simulink model "tb_lv_rails"  (R2026b)
model workspace (MAT data in the model file):
  TB.vaux_t = [0 10000000]
  TB.vaux_v = [52 52]
  TB.P24_t = [0 10000000]
  TB.P24_v = [53 53]
  TB.P12_t = [0 10000000]
  TB.P12_v = [99 99]
  TB.P5_t = [0 10000000]
  TB.P5_v = [2.5 2.5]
  TB.P3_t = [0 10000000]
  TB.P3_v = [0.6 0.6]
  TB.fan_t = [0 10000000]
  TB.fan_v = [0 0]
  TB.k3_t = [0 10000000]
  TB.k3_v = [0 0]
  TB.imp_R = 1000
  TB.MaxNonlinIter = 3
  TB.MaxModeIter = 2
undefined symbols (not defined in the file or in its folder): Ts
libraries: fl_lib x4, nesl_utility x4, simulink x1, ee_lib x1
settings Model: Creator=aomar  LastModifiedBy=aomar

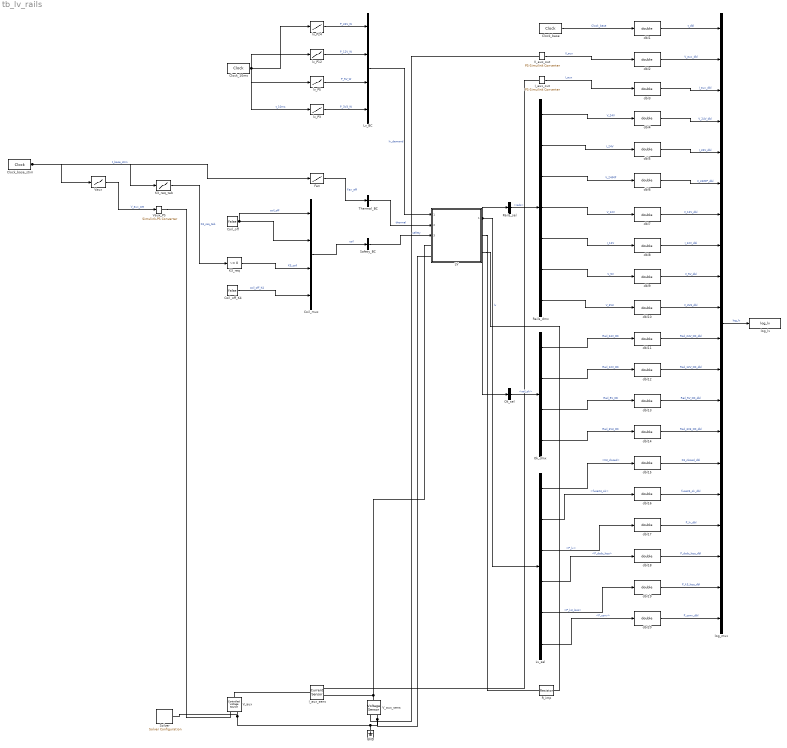
== system tb_lv_rails ==
  Clock_10ms : DigitalClock  SampleTime=Ts.ctrl
  Clock_base : DigitalClock  SampleTime=Ts.base
  Clock_base_stim : DigitalClock  SampleTime=Ts.base
  Coil_mux : Mux
  Coil_off : Constant  Value=false  OutDataTypeStr=boolean  SampleTime=Ts.base
  Coil_off_K4 : Constant  Value=false  OutDataTypeStr=boolean  SampleTime=Ts.base
  Fan : Lookup_n-D  NumberOfTableDimensions=1  BreakpointsForDimension1=TB.fan_t  Table=TB.fan_v  InterpMethod=Flat  ExtrapMethod=Clip  InternalRulePriority=Speed  RndMeth=Simplest
  GND : fl_lib/Electrical/Electrical Elements/Electrical Reference
  I_aux_out : nesl_utility/PS-Simulink Converter  PhysicalDomain=network_engine_domain  SubClassName=ps_output  LeftPortType=input  RightPortType=output  PseudoPeriodic=off  Frequencies=[]  VectorFormat=inherit  Unit=A  AffineConversion=off
  I_aux_sens : fl_lib/Electrical/Electrical Sensors/Current Sensor
  K3_req : simulink/Logic and Bit Operations/Compare To Zero  relop=~=  OutDataTypeStr=boolean
  K3_req_tab : Lookup_n-D  NumberOfTableDimensions=1  BreakpointsForDimension1=TB.k3_t  Table=TB.k3_v  InterpMethod=Flat  ExtrapMethod=Clip  InternalRulePriority=Speed  RndMeth=Simplest
  LV : Subsystem  ReferencedSubsystem=LV_Distribution
  Lv_BC : BusCreator  Inputs=4  OutDataTypeStr=Bus: Bus_LV_LoadDemand  NonVirtualBus=on
      settings: InheritFromInputs=off
  Lv_sel : BusSelector  OutputSignals=K3_closed,fuse24_ok,P_lv,P_dcdc_loss,P_k3_loss,P_conv
  Ok_dmx : Demux
  Ok_sel : BusSelector  OutputSignals=rail_ok
  R_imp : ee_lib/Passive/Resistor  R=TB.imp_R Ohm  enable_R_tol=ee.enum.toleranceApplication.none  R_tol=5  tol_distribution=ee.enum.toleranceDistribution.uniform  nSigma=4  enable_operating_limits=ee.enum.enable.no  operating_limit_action=ee.enum.passive.reportOpLim.warn  power_rating=1 W  max_working_voltage=100 V  noise_mode=ee.enum.sources.noise.Disabled  Tdevice=25 degC  sample_time=1e-3 s  repeatability=ee.enum.ic.repeatability.notRepeatable  user_seed=0  auto_seed=1503454846  power_derating_T1=70 degC  power_derating_T2=155 degC  operating_temperature_range_vec=[-50, 150] degC  alpha=3.93e-3 1/K  Tmeas=25 degC  thermal_mass=100 J/K  temperature_specify=off  temperature_priority=High  temperature=298.15 K  temperature_nominal_specify=off  temperature_nominal_value=1  temperature_nominal_unit=K
  Rails_dmx : Demux  Outputs=7
  Rails_sel : BusSelector  OutputSignals=rails
  Safety_BC : BusCreator  Inputs=1
  Solver : nesl_utility/Solver Configuration  PhysicalDomain=network_engine_domain  SubClassName=solver  LeftPortType=input  RightPortType=generic  Tones=[]  Harmonics=[]  SimulateNoise=off  Profile=off  UseLocalSampling=off  EnableSwitchedLinearOptims=on  FrequencyDomain=off  UseCCode=off  RelTol=0.001  AbsTol=0.001  MinStep=1e-09  ToWorkspace=off  RevertToSquareIcSolve=off  NumHomotopyIterations=100  PhasorMode=off  PhasorModeNumHarmonics=1  ConsistencySolver=NEWTON_XTOL_AFTER_FTOL  CanonicalOrdering=CANONICAL  OptimizeIntermediates=OPTIMIZED  MulticoreSolverChoice=BACKWARD_EULER  IndexReductionMethod=DerivativeReplacement  DoDC=off  ResidualTolerance=1e-09  ConsistencyTolSource=GLOBAL  ConsistencyAbsTol=0.001  ConsistencyRelTol=0.001  ConsistencyTolFactor=0.001  UseLocalSolver=on  LocalSolverChoice=NE_BACKWARD_EULER_ADVANCER  ResolveIndetEquations=on  FunctionEvalNumThread=1  LocalSolverSampleTime=P.sim.ssc.Ts  DoFixedCost=on  MaxNonlinIter=TB.MaxNonlinIter  MaxModeIter=TB.MaxModeIter  ComputeImpulses=off  ImpulseIterations=2  LinearAlgebra=auto  LinearAlgebraNumThread=0  EquationFormulation=NE_TIME_EF  DelaysMemoryBudget=1024  AutomaticFiltering=on  FilteringTimeConstant=0.001  PartitionStorageMethod=AS_NEEDED  PartitionMemoryBudget=1024  PartitionMethod=BALANCED  MultibodyUseLocalSolver=off  MultibodyLocalSolverChoice=ODE1  MultibodyLocalSolverSampleTime=0.001
  Thermal_BC : BusCreator  Inputs=1
  V_aux : fl_lib/Electrical/Electrical Sources/Controlled Voltage Source
  V_aux_out : nesl_utility/PS-Simulink Converter  PhysicalDomain=network_engine_domain  SubClassName=ps_output  LeftPortType=input  RightPortType=output  PseudoPeriodic=off  Frequencies=[]  VectorFormat=inherit  Unit=V  AffineConversion=off
  V_aux_sens : fl_lib/Electrical/Electrical Sensors/Voltage Sensor
  Vaux : Lookup_n-D  NumberOfTableDimensions=1  BreakpointsForDimension1=TB.vaux_t  Table=TB.vaux_v  ExtrapMethod=Clip  InternalRulePriority=Speed  RndMeth=Simplest
  Vaux_PS : nesl_utility/Simulink-PS Converter  PhysicalDomain=network_engine_domain  SubClassName=ps_input  LeftPortType=input  RightPortType=output  PseudoPeriodic=off  Frequencies=[]  NoiseDistribution=none  NoiseParameters=[]  Unit=V  AffineConversion=off  FilteringAndDerivatives=zero  SimscapeFilterOrder=1  InputFilterTimeConstant=0.001  UdotUserProvided=0
  dbl{1..20} (20 alike) : DataTypeConversion  OutDataTypeStr=double  SaturateOnIntegerOverflow=off  RndMeth=Floor
  log_lv : ToWorkspace  VariableName=log_lv  SampleTime=-1
  log_mux : Mux  Inputs=20
  lv_P12 : Lookup_n-D  NumberOfTableDimensions=1  BreakpointsForDimension1=TB.P12_t  Table=TB.P12_v  InterpMethod=Flat  ExtrapMethod=Clip  InternalRulePriority=Speed  RndMeth=Simplest
  lv_P24 : Lookup_n-D  NumberOfTableDimensions=1  BreakpointsForDimension1=TB.P24_t  Table=TB.P24_v  InterpMethod=Flat  ExtrapMethod=Clip  InternalRulePriority=Speed  RndMeth=Simplest
  lv_P3 : Lookup_n-D  NumberOfTableDimensions=1  BreakpointsForDimension1=TB.P3_t  Table=TB.P3_v  InterpMethod=Flat  ExtrapMethod=Clip  InternalRulePriority=Speed  RndMeth=Simplest
  lv_P5 : Lookup_n-D  NumberOfTableDimensions=1  BreakpointsForDimension1=TB.P5_t  Table=TB.P5_v  InterpMethod=Flat  ExtrapMethod=Clip  InternalRulePriority=Speed  RndMeth=Simplest
  wires:
  Clock_base_stim/1 -> K3_req_tab/1, Vaux/1, Fan/1  "t_base_stim"
  Vaux/1 -> Vaux_PS/1  "V_aux_set"
  K3_req_tab/1 -> K3_req/1  "K3_req_tab"
  Coil_off/1 -> Coil_mux/2, Coil_mux/1  "coil_off"
  Coil_off_K4/1 -> Coil_mux/4  "coil_off_K4"
  K3_req/1 -> Coil_mux/3  "K3_coil"
  Clock_10ms/1 -> lv_P24/1, lv_P3/1, lv_P12/1, lv_P5/1  "t_10ms"
  Coil_mux/1 -> Safety_BC/1  "coil"
  lv_P24/1 -> Lv_BC/1  "P_24V_W"
  lv_P12/1 -> Lv_BC/2  "P_12V_W"
  lv_P5/1 -> Lv_BC/3  "P_5V_W"
  lv_P3/1 -> Lv_BC/4  "P_3V3_W"
  Fan/1 -> Thermal_BC/1  "Fan_eff"
  Lv_BC/1 -> LV/1  "lv_demand"
  Thermal_BC/1 -> LV/2  "thermal"
  Safety_BC/1 -> LV/3  "safety"
  LV/1 -> Lv_sel/1, Ok_sel/1, Rails_sel/1  "lv"
  Rails_sel/1 -> Rails_dmx/1  "<rails>"
  Ok_sel/1 -> Ok_dmx/1  "<rail_ok>"
  Rails_dmx/1 -> dbl4/1  "V_24V"
  Rails_dmx/2 -> dbl5/1  "I_24V"
  Rails_dmx/3 -> dbl6/1  "V_24IMP"
  Rails_dmx/4 -> dbl7/1  "V_12V"
  Rails_dmx/5 -> dbl8/1  "I_12V"
  Rails_dmx/6 -> dbl9/1  "V_5V"
  Rails_dmx/7 -> dbl10/1  "V_3V3"
  Ok_dmx/1 -> dbl11/1  "Rail_24V_OK"
  Ok_dmx/2 -> dbl12/1  "Rail_12V_OK"
  Ok_dmx/3 -> dbl13/1  "Rail_5V_OK"
  Ok_dmx/4 -> dbl14/1  "Rail_3V3_OK"
  Lv_sel/1 -> dbl15/1  "<K3_closed>"
  Lv_sel/2 -> dbl16/1  "<fuse24_ok>"
  Lv_sel/3 -> dbl17/1  "<P_lv>"
  Lv_sel/4 -> dbl18/1  "<P_dcdc_loss>"
  Lv_sel/5 -> dbl19/1  "<P_k3_loss>"
  Lv_sel/6 -> dbl20/1  "<P_conv>"
  V_aux_out/1 -> dbl2/1  "V_aux"
  I_aux_out/1 -> dbl3/1  "I_aux"
  Clock_base/1 -> dbl1/1  "Clock_base"
  dbl1/1 -> log_mux/1  "t_dbl"
  dbl2/1 -> log_mux/2  "V_aux_dbl"
  dbl3/1 -> log_mux/3  "I_aux_dbl"
  dbl4/1 -> log_mux/4  "V_24V_dbl"
  dbl5/1 -> log_mux/5  "I_24V_dbl"
  dbl6/1 -> log_mux/6  "V_24IMP_dbl"
  dbl7/1 -> log_mux/7  "V_12V_dbl"
  dbl8/1 -> log_mux/8  "I_12V_dbl"
  dbl9/1 -> log_mux/9  "V_5V_dbl"
  dbl10/1 -> log_mux/10  "V_3V3_dbl"
  dbl11/1 -> log_mux/11  "Rail_24V_OK_dbl"
  dbl12/1 -> log_mux/12  "Rail_12V_OK_dbl"
  dbl13/1 -> log_mux/13  "Rail_5V_OK_dbl"
  dbl14/1 -> log_mux/14  "Rail_3V3_OK_dbl"
  dbl15/1 -> log_mux/15  "K3_closed_dbl"
  dbl16/1 -> log_mux/16  "fuse24_ok_dbl"
  dbl17/1 -> log_mux/17  "P_lv_dbl"
  dbl18/1 -> log_mux/18  "P_dcdc_loss_dbl"
  dbl19/1 -> log_mux/19  "P_k3_loss_dbl"
  dbl20/1 -> log_mux/20  "P_conv_dbl"
  log_mux/1 -> log_lv/1  "log_lv"
  connections:
  I_aux_out/LConn1 -- I_aux_sens/RConn1
  V_aux/LConn1 -- I_aux_sens/LConn1
  V_aux_sens/LConn1 -- LV/LConn1 -- I_aux_sens/RConn2
  LV/RConn1 -- R_imp/LConn1
  LV/RConn2 -- R_imp/RConn1
  Vaux_PS/RConn1 -- V_aux/RConn1
  V_aux_sens/RConn2 -- LV/LConn2 -- GND/LConn1 -- V_aux/RConn2 -- Solver/RConn1
  V_aux_out/LConn1 -- V_aux_sens/RConn1
